simulink model "buck"  (R2022b)
settings: Solver=ode4  StartTime=0.0  StopTime=0.005  FixedStep=Ts  RelTol=1e-3
InitFcn:
  | buck_init
values from neighbouring files (symbols this model uses):
  Ts = 1e-8    (= 1e-08)    [buck_init.m]
libraries: spsSeriesRLCBranchLib x6, peripheral_utilities x4, spsControlledVoltageSourceLib x1, spsGroundLib x1, spspowerguiLib x1
settings Model: Creator=javnson  LastModifiedBy=javnson

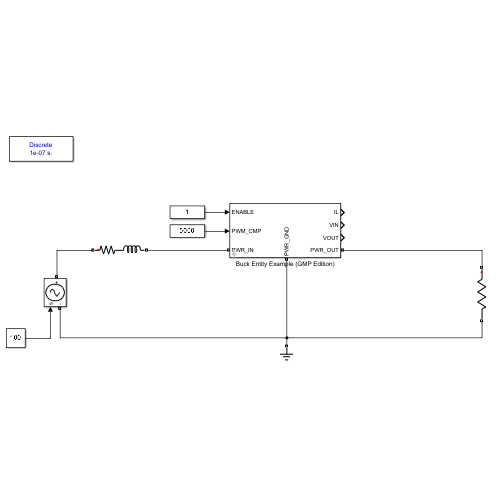
[thumbnail: Simulink's stored preview of the top-level diagram]
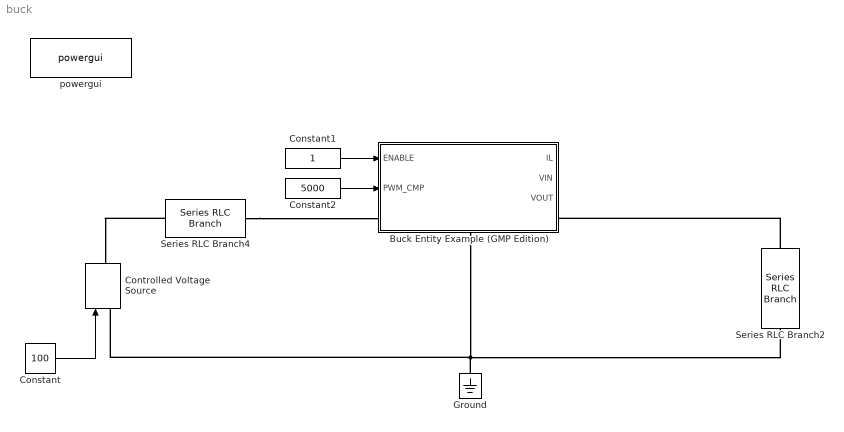
== system buck ==
  Buck Entity Example (GMP Edition) : Subsystem  mask{Cin=100e-6, Cout=100e-6, L=50e-6, RL=1e-3, RCin=0.1, RCout=100e-6, Cout2=1e-6, RCout2=1e-4, Voadc_bias=0, Voadc_fs=120, ADC_RES=16, Viadc_fs=120, Viadc_bias=0, Iladc_fs=60, Iadc_bias=30, fswitch=30e3, CMP_MAX=10000, DB_UP=100, DB_DW=100, Rds_on=0.02, Lon=0, Rd=0.01, Vf=0.3, Rs=1e5, Cs=inf}
      settings: PortSchema="{\"entries\":[{\"content\":{\"sides\":[{\"content\":{\"connectorIds\":[\"In1\",\"In2\",\"LConn1\"]},\"type\":\"ConnectorPlacement.EquallySpacedRectSide\",\"uuid\":\"3dc1f0aa-256b-4eee-9ab4-ff52cb056450\"},{\"content\":{\"connectorIds\":[\"Out1\",\"Out2\",\"Out3\",\"RConn1\"],\"side\":\"RIGHT\"},\"type\":\"ConnectorPlacement.EquallySpacedRectSide\",\"uuid\":\"c182f68c-961e-48e9-b450-8a2d07cca989\"},{\"content\":{\"connectorIds\":[],\"side\":\"TOP\"},\"type\":\"ConnectorPlacement.EquallySpacedRectSide\",\"uuid\":\"77cafdf0-ba99-4ec6-a003-27712a389068\"},{\"content\":{\"connectorIds\":[\"RConn2\"],\"side\":\"BOTTOM\"},\"type\":\"ConnectorPlacement.EquallySpacedRectSide\",\"uuid\":\"1cb5a4dc-5d4b-4bbe-a9bd-2c66268ddaed\"}]},\"type\":\"ConnectorPlacement.EquallySpacedConnector\",\"uuid\":\"ec8c1d3d-5436-4386-91dc-89cedd685bc0\"}],\"packageUris\":[\"http://schema.mathworks.com/mf0/Connector/R2020b\"],\"version\":\"1.0\"}"
      mask DialogControl Container4 Prompt: Main Circuit
      mask DialogControl Control2 Prompt: Input port Capacitor, unit F
      mask DialogControl Control3 Prompt: Ouput port Capacitor, unit F
      mask DialogControl Control4 Prompt: Filter Inductor, unit H
      mask DialogControl Container6 Prompt: Other Parameters
      mask DialogControl Control5 Prompt: Resistance of Inductor, unit Ohm
      mask DialogControl Control9 Prompt: Resistance of input Capacitor, unit Ohm
      mask DialogControl Control6 Prompt: Resistance of output Capacitor, unit Ohm
      mask DialogControl Control7 Prompt: Low resistance output Capacitor branch, Capacitor, unit F
      mask DialogControl Control8 Prompt: Low resistance output capacitor branch, resistance of capacitor, unit Ohm
      mask DialogControl Container5 Prompt: Sensor
      mask DialogControl Control15 Prompt: Output Voltage ADC, Bias Voltage, unit V
      mask DialogControl Control14 Prompt: Output Voltage ADC, Full Scale Voltage, unit V
      mask DialogControl Control10 Prompt: ADC resolution, bits
      mask DialogControl Control11 Prompt: Input Voltage ADC, Full Scale Voltage, unit V
      mask DialogControl Control12 Prompt: Input Voltage ADC, Bias Voltage, unit V
      mask DialogControl Control13 Prompt: Indctor Current ADC, Full Scale, unit A
      mask DialogControl Control16 Prompt: Inductor Current ADC, Bias Current, unit A
      mask DialogControl Container7 Prompt: PWM Modulator
      mask DialogControl Control17 Prompt: PWM frequency, unit Hz
      mask DialogControl Control18 Prompt: Full Scale PWM Compare value
      mask DialogControl Control19 Prompt: Deadband Setting
      mask DialogControl Container8 Prompt: MOSFET
      mask DialogControl Control20 Prompt: Rds(on), unit Ohm
      mask DialogControl Control21 Prompt: Internal diode inductance, unit H
      mask DialogControl Control22 Prompt: Internal diode resistance Rd, unit Ohm
      mask DialogControl Control23 Prompt: Internal diode forward voltage Vf, unit V
      mask DialogControl Control24 Prompt: Snubber resistance Rs, unit Ohm
      mask DialogControl Control25 Prompt: Snubber Capacitance Cs, unit F
  Constant : Constant  Value=100
  Constant1 : Constant
  Constant2 : Constant  Value=5000
  Controlled Voltage Source : spsControlledVoltageSourceLib/Controlled Voltage Source  Initialize=on  Source_Type=AC  Amplitude=0  Phase=0  Frequency=0  Measurements=None
  Ground : spsGroundLib/Ground  LConnTagsString=a
  Series RLC Branch2 : spsSeriesRLCBranchLib/Series RLC Branch  LConnTagsString=__new0  RConnTagsString=__new0  BranchType=R  Resistance=15  Inductance=50e-6  SetiL0=off  InitialCurrent=0  Capacitance=1e-6  Setx0=off  InitialVoltage=0  Measurements=None
  Series RLC Branch4 : spsSeriesRLCBranchLib/Series RLC Branch  LConnTagsString=__new0  RConnTagsString=__new0  BranchType=RL  Resistance=1e-3  Inductance=10e-6  SetiL0=off  InitialCurrent=0  Capacitance=1e-6  Setx0=off  InitialVoltage=0  Measurements=None
  powergui : spspowerguiLib/powergui  Priority=1  SimulationMode=Discrete  SampleTime=Ts  frequency=60  Iterations=50  frequencyindice=0  Pbase=100e6  ErrMax=1e-4  UnitsV=kV  UnitsW=MW  buscounter=0  FunctionMessages=off  echomessages=off  EnableUseOfTLC=off  CurrentSourceSwitches=off  DisableSnubberDevices=off  DisableRonSwitches=off  DisableVfSwitches=off  DisplayEquations=off  AutomaticDiscreteSolvers=off  SolverType=Tustin/Backward Euler (TBE)  Interpol=off  ExternalGateDelay=off  methode=off  Ts=100  x0status=blocks  SPID=on  SwTol=0  HookPort=off  NonlinearTolerance=1e-4  nMaxIteration=100  ContinueOnMaxIteration=off  RestoreLinks=warning  ResistiveCurrentMeasurement=off  Frange=[0:2:500]  Ylog=off  Xlog=on  ShowGrid=off  save=off  variable=ZData  structure=0  ZoomFFT=off  StartTime=0.0  cycles=1  DisplayStyle=1  fundamental=60  FreqAxis=off  MaxFrequency=1000  frequencyindicesteady=1  RmsSteady=1  display=off
  wires:
  Constant/1 -> Controlled Voltage Source/1
  Constant1/1 -> Buck Entity Example (GMP Edition)/1(ENABLE)
  Constant2/1 -> Buck Entity Example (GMP Edition)/2(PWM_CMP)
  connections:
  Series RLC Branch4/LConn1 -- Controlled Voltage Source/RConn1
  Buck Entity Example (GMP Edition)/RConn2 -- Ground/LConn1 -- Series RLC Branch2/RConn1 -- Controlled Voltage Source/LConn1
  Series RLC Branch4/RConn1 -- Buck Entity Example (GMP Edition)/LConn1
  Series RLC Branch2/LConn1 -- Buck Entity Example (GMP Edition)/RConn1

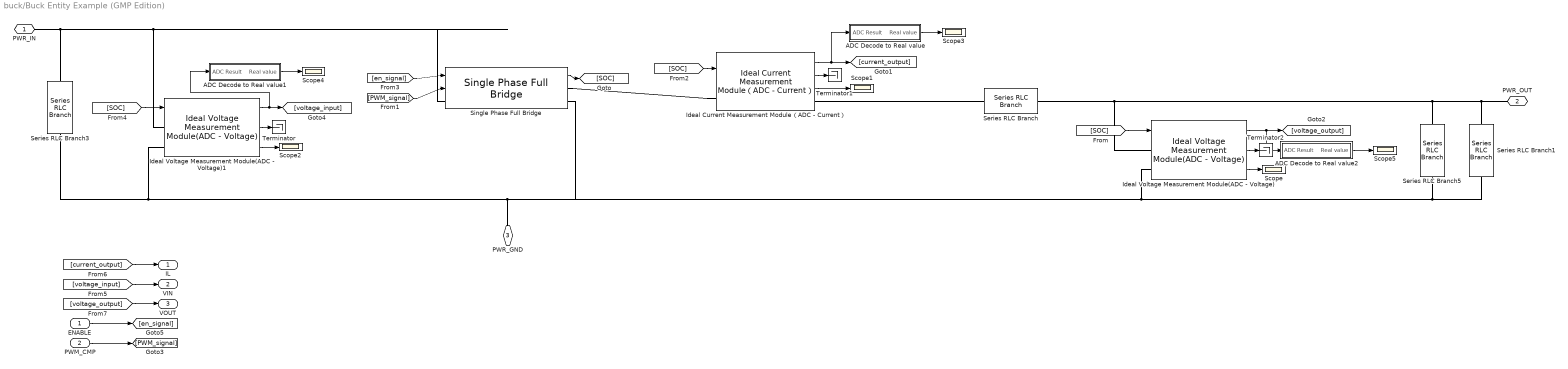
== system buck/Buck Entity Example (GMP Edition) ==
  ENABLE : Inport
  PWM_CMP : Inport  Port=2
  ADC Decode to Real value : Subsystem  mask{ADC_GAIN=1, ADC_BIT=16, ADC_REF=60, ADC_BIAS=30}
      settings: CopyFcn=set_param(gcbh,'LinkStatus','none');
      mask DialogControl DescGroupVar Prompt: ADC Decoder
      mask DialogControl DescTextVar Prompt: GMP CTL Simulink Utilities: virtual peripherals
      mask DialogControl Control2 Prompt: Transfer adc sample result to real value.
      mask DialogControl ParameterGroupVar Prompt: 参数
      mask DialogControl Control3 Prompt: ADC Voltage Gain (Scale Factor):
      mask DialogControl Control4 Prompt: ADC resolution:
      mask DialogControl Control5 Prompt: ADC reference Voltage (V), when ADC_GAIN=1, ADC_REF = ADC full scale
      mask DialogControl Control6 Prompt: ADC Bias Voltage(V)
  ADC Decode to Real value1 : Subsystem  mask{ADC_GAIN=1, ADC_BIT=16, ADC_REF=120, ADC_BIAS=0}
      settings: CopyFcn=set_param(gcbh,'LinkStatus','none');
      mask DialogControl DescGroupVar Prompt: ADC Decoder
      mask DialogControl DescTextVar Prompt: GMP CTL Simulink Utilities: virtual peripherals
      mask DialogControl Control2 Prompt: Transfer adc sample result to real value.
      mask DialogControl ParameterGroupVar Prompt: 参数
      mask DialogControl Control3 Prompt: ADC Voltage Gain (Scale Factor):
      mask DialogControl Control4 Prompt: ADC resolution:
      mask DialogControl Control5 Prompt: ADC reference Voltage (V), when ADC_GAIN=1, ADC_REF = ADC full scale
      mask DialogControl Control6 Prompt: ADC Bias Voltage(V)
  ADC Decode to Real value2 : Subsystem  mask{ADC_GAIN=1, ADC_BIT=16, ADC_REF=120, ADC_BIAS=0}
      settings: CopyFcn=set_param(gcbh,'LinkStatus','none');
      mask DialogControl DescGroupVar Prompt: ADC Decoder
      mask DialogControl DescTextVar Prompt: GMP CTL Simulink Utilities: virtual peripherals
      mask DialogControl Control2 Prompt: Transfer adc sample result to real value.
      mask DialogControl ParameterGroupVar Prompt: 参数
      mask DialogControl Control3 Prompt: ADC Voltage Gain (Scale Factor):
      mask DialogControl Control4 Prompt: ADC resolution:
      mask DialogControl Control5 Prompt: ADC reference Voltage (V), when ADC_GAIN=1, ADC_REF = ADC full scale
      mask DialogControl Control6 Prompt: ADC Bias Voltage(V)
  Ideal Current Measurement Module（ADC - Current） : peripheral_utilities/Ideal Current Measurement Module（ADC - Current）  ADC_GAIN=1  ADC_BIT=ADC_RES  ADC_REFERENCE=Iladc_fs  ADC_BIAS=Iadc_bias  ADC_INIT=0
      settings: SourceProductName=GMP Utilities Library
  Ideal Voltage Measurement Module(ADC - Voltage) : peripheral_utilities/Ideal Voltage Measurement Module(ADC - Voltage)  ADC_GAIN=1  ADC_BIT=ADC_RES  ADC_REFERENCE=Voadc_fs  ADC_BIAS=Voadc_bias  ADC_INIT=0
      settings: SourceProductName=GMP Utilities Library
  Ideal Voltage Measurement Module(ADC - Voltage)1 : peripheral_utilities/Ideal Voltage Measurement Module(ADC - Voltage)  ADC_GAIN=1  ADC_BIT=ADC_RES  ADC_REFERENCE=Viadc_fs  ADC_BIAS=Viadc_bias  ADC_INIT=0
      settings: SourceProductName=GMP Utilities Library
  Scope{,1..5} (6 alike) : Scope
  Series RLC Branch : spsSeriesRLCBranchLib/Series RLC Branch  LConnTagsString=__new0  RConnTagsString=__new0  BranchType=RL  Resistance=RL  Inductance=L  SetiL0=off  InitialCurrent=0  Capacitance=1e-6  Setx0=off  InitialVoltage=0  Measurements=None
  Series RLC Branch1 : spsSeriesRLCBranchLib/Series RLC Branch  LConnTagsString=__new0  RConnTagsString=__new0  BranchType=RC  Resistance=RCout2  Inductance=50e-6  SetiL0=off  InitialCurrent=0  Capacitance=Cout2  Setx0=off  InitialVoltage=0  Measurements=None
  Series RLC Branch3 : spsSeriesRLCBranchLib/Series RLC Branch  LConnTagsString=__new0  RConnTagsString=__new0  BranchType=RC  Resistance=RCin  Inductance=50e-6  SetiL0=off  InitialCurrent=0  Capacitance=Cin  Setx0=off  InitialVoltage=0  Measurements=None
  Series RLC Branch5 : spsSeriesRLCBranchLib/Series RLC Branch  LConnTagsString=__new0  RConnTagsString=__new0  BranchType=RC  Resistance=RCout  Inductance=50e-6  SetiL0=off  InitialCurrent=0  Capacitance=Cout  Setx0=off  InitialVoltage=0  Measurements=None
  Single Phase Full Bridge : peripheral_utilities/Single Phase Full Bridge  fswitch=fswitch  CMP_MAX=CMP_MAX  Deadband_Upper=DB_UP  Deadband_Lower=DB_DW  phase_shift=0  R_mosfet_on=Rds_on  Lon=Lon  Rd=Rd  Vf=Vf  Rs=Rs  Cs=Cs
      settings: SourceProductName=GMP Utilities Library
  Terminator : Terminator
  Terminator1 : Terminator
  Terminator2 : Terminator
  PWR_IN : PMIOPort  Side=Left
  PWR_OUT : PMIOPort  Port=2  Side=Right
  PWR_GND : PMIOPort  Port=3  Side=Right
  IL : Outport
  VIN : Outport  Port=2
  VOUT : Outport  Port=3
  wires:
  [PWM_signal] -> Single Phase Full Bridge/2
  [SOC] -> Ideal Current Measurement Module（ADC - Current）/1
  Ideal Current Measurement Module（ADC - Current）/1 -> ADC Decode to Real value/1(ADC Result), [current_output]
  Ideal Voltage Measurement Module(ADC - Voltage)1/1 -> ADC Decode to Real value1/1(ADC Result), [voltage_input]
  Ideal Voltage Measurement Module(ADC - Voltage)/3 -> Scope/1
  Ideal Voltage Measurement Module(ADC - Voltage)/1 -> ADC Decode to Real value2/1(ADC Result), [voltage_output]
  [voltage_output] -> VOUT/1
  ENABLE/1 -> [en_signal]
  Ideal Current Measurement Module（ADC - Current）/3 -> Scope1/1
  Ideal Voltage Measurement Module(ADC - Voltage)1/3 -> Scope2/1
  [SOC] -> Ideal Voltage Measurement Module(ADC - Voltage)1/1
  Ideal Current Measurement Module（ADC - Current）/2 -> Terminator1/1
  [SOC] -> Ideal Voltage Measurement Module(ADC - Voltage)/1
  Single Phase Full Bridge/1 -> [SOC]
  PWM_CMP/1 -> [PWM_signal]
  ADC Decode to Real value2/1(Real value) -> Scope5/1
  [en_signal] -> Single Phase Full Bridge/1
  ADC Decode to Real value/1(Real value) -> Scope3/1
  ADC Decode to Real value1/1(Real value) -> Scope4/1
  Ideal Voltage Measurement Module(ADC - Voltage)/2 -> Terminator2/1
  Ideal Voltage Measurement Module(ADC - Voltage)1/2 -> Terminator/1
  [current_output] -> IL/1
  [voltage_input] -> VIN/1
  connections:
  Ideal Current Measurement Module（ADC - Current）/RConn1 -- Series RLC Branch/LConn1
  Series RLC Branch3/LConn1 -- PWR_IN/RConn1 -- Ideal Voltage Measurement Module(ADC - Voltage)1/LConn1 -- Single Phase Full Bridge/LConn1
  Ideal Current Measurement Module（ADC - Current）/LConn1 -- Single Phase Full Bridge/RConn1
  Series RLC Branch1/LConn1 -- PWR_OUT/RConn1 -- Series RLC Branch5/LConn1 -- Ideal Voltage Measurement Module(ADC - Voltage)/LConn1 -- Series RLC Branch/RConn1
  Ideal Voltage Measurement Module(ADC - Voltage)1/LConn2 -- PWR_GND/RConn1 -- Series RLC Branch1/RConn1 -- Series RLC Branch5/RConn1 -- Ideal Voltage Measurement Module(ADC - Voltage)/LConn2 -- Single Phase Full Bridge/RConn2 -- Series RLC Branch3/RConn1

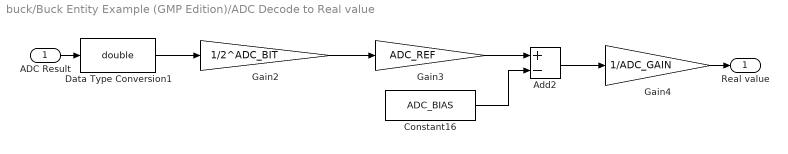
== system buck/Buck Entity Example (GMP Edition)/ADC Decode to Real value ==
  ADC Result : Inport
  Add2 : Sum  Inputs=+-
  Constant16 : Constant  Value=ADC_BIAS
  Data Type Conversion1 : DataTypeConversion  OutDataTypeStr=double  SaturateOnIntegerOverflow=off  RndMeth=Floor
  Gain2 : Gain  Gain=1/2^ADC_BIT
  Gain3 : Gain  Gain=ADC_REF
  Gain4 : Gain  Gain=1/ADC_GAIN
  Real value : Outport
  wires:
  ADC Result/1 -> Data Type Conversion1/1
  Gain2/1 -> Gain3/1
  Constant16/1 -> Add2/2
  Gain4/1 -> Real value/1
  Add2/1 -> Gain4/1
  Gain3/1 -> Add2/1
  Data Type Conversion1/1 -> Gain2/1

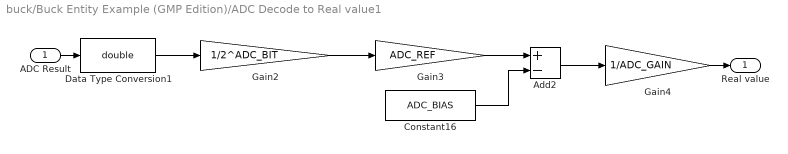
== system buck/Buck Entity Example (GMP Edition)/ADC Decode to Real value1 ==
  ADC Result : Inport
  Add2 : Sum  Inputs=+-
  Constant16 : Constant  Value=ADC_BIAS
  Data Type Conversion1 : DataTypeConversion  OutDataTypeStr=double  SaturateOnIntegerOverflow=off  RndMeth=Floor
  Gain2 : Gain  Gain=1/2^ADC_BIT
  Gain3 : Gain  Gain=ADC_REF
  Gain4 : Gain  Gain=1/ADC_GAIN
  Real value : Outport
  wires:
  ADC Result/1 -> Data Type Conversion1/1
  Gain2/1 -> Gain3/1
  Constant16/1 -> Add2/2
  Gain4/1 -> Real value/1
  Add2/1 -> Gain4/1
  Gain3/1 -> Add2/1
  Data Type Conversion1/1 -> Gain2/1

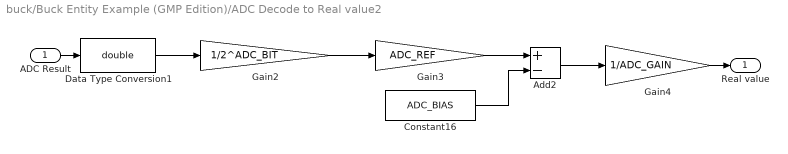
== system buck/Buck Entity Example (GMP Edition)/ADC Decode to Real value2 ==
  ADC Result : Inport
  Add2 : Sum  Inputs=+-
  Constant16 : Constant  Value=ADC_BIAS
  Data Type Conversion1 : DataTypeConversion  OutDataTypeStr=double  SaturateOnIntegerOverflow=off  RndMeth=Floor
  Gain2 : Gain  Gain=1/2^ADC_BIT
  Gain3 : Gain  Gain=ADC_REF
  Gain4 : Gain  Gain=1/ADC_GAIN
  Real value : Outport
  wires:
  ADC Result/1 -> Data Type Conversion1/1
  Gain2/1 -> Gain3/1
  Constant16/1 -> Add2/2
  Gain4/1 -> Real value/1
  Add2/1 -> Gain4/1
  Gain3/1 -> Add2/1
  Data Type Conversion1/1 -> Gain2/1
